simulink model "ex1s"  (R2022a)
settings: Solver=VariableStepAuto  StartTime=0.0  StopTime=10.0  RelTol=1e-3
settings Model: Creator=giova  LastModifiedBy=giova

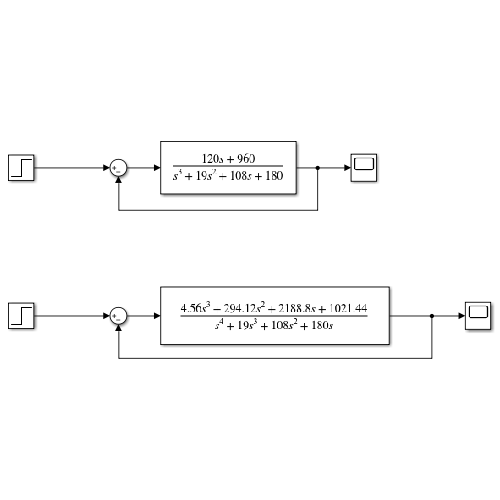
[thumbnail: Simulink's stored preview of the top-level diagram]
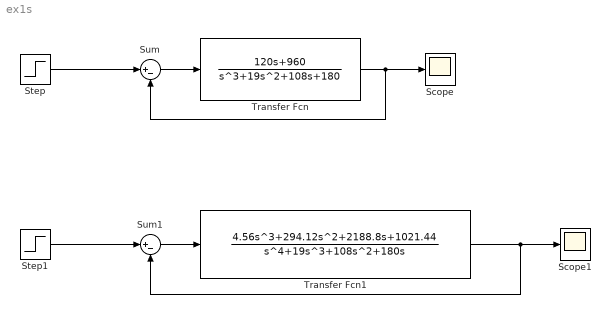
== system ex1s ==
  Scope : Scope
  Scope1 : Scope
  Step : Step  SampleTime=0
  Step1 : Step  SampleTime=0
  Sum : Sum  Inputs=|+-
  Sum1 : Sum  Inputs=|+-
  Transfer Fcn : TransferFcn  Numerator=[120 960]  Denominator=[1 19 108 180]
  Transfer Fcn1 : TransferFcn  Numerator="[4.56  294.12  2188.8  1021.44]"  Denominator="[1  19  108  180  0]"
  wires:
  Step/1 -> Sum/1
  Sum/1 -> Transfer Fcn/1
  Transfer Fcn/1 -> Sum/2, Scope/1
  Transfer Fcn1/1 -> Sum1/2, Scope1/1
  Step1/1 -> Sum1/1
  Sum1/1 -> Transfer Fcn1/1
